simulink model "backflow_test"  (R2024b)
settings: Solver=FixedStepDiscrete  StartTime=0.0  StopTime=600  FixedStep=0.0002  RelTol=1e-3
InitFcn:
  |    parameters_charlton;
  |    parameters_ferreira;
  |    parameters_backflowcontrol;
undefined symbols (not defined in the file): A_tank, DiscIntNeverNeededParam, H_REF_MAX, H_REF_MIN, HR, Ki_fb, Kp_fb, LUT_Q, LUT_u, N, Ts, U_FB_MAX
libraries: slpidlib x2, simulink x1
settings Model: Creator=sammy  LastModifiedBy=sammy

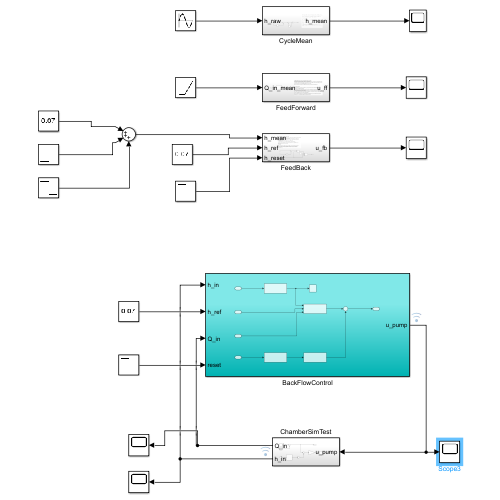
[thumbnail: Simulink's stored preview of the top-level diagram]
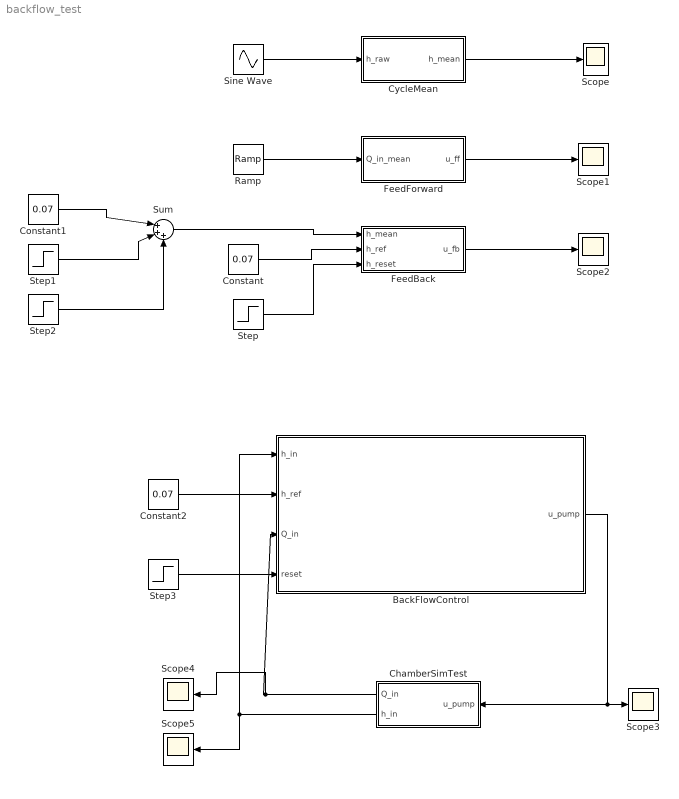
== system backflow_test ==
  BackFlowControl : Subsystem
  ChamberSimTest : Subsystem
  Constant : Constant  Value=0.07
  Constant1 : Constant  Value=0.07
  Constant2 : Constant  Value=0.07
  CycleMean : Subsystem
  FeedBack : Subsystem
  FeedForward : Subsystem
  Ramp : simulink/Sources/Ramp  slope=10  start=0  InitialOutput=0
  Scope{,1..5} (6 alike) : Scope
  Sine Wave : Sin  Amplitude=10  Frequency=2*pi*HR/60  SampleTime=0
  Step : Step  Time=5  Before=1  After=0  SampleTime=0
  Step1 : Step  Time=10  After=0.02  SampleTime=0
  Step2 : Step  Time=70  After=-0.02  SampleTime=0
  Step3 : Step  Time=5  Before=1  After=0  SampleTime=0
  Sum : Sum  Inputs=|+++
  wires:
  Sine Wave/1 -> CycleMean/1(h_raw)
  CycleMean/1(h_mean) -> Scope/1
  Ramp/1 -> FeedForward/1(Q_in_mean)
  FeedForward/1(u_ff) -> Scope1/1
  Step/1 -> FeedBack/3(h_reset)
  Constant/1 -> FeedBack/2(h_ref)
  Sum/1 -> FeedBack/1(h_mean)
  Constant1/1 -> Sum/1
  Step1/1 -> Sum/2
  Step2/1 -> Sum/3
  FeedBack/1(u_fb) -> Scope2/1
  BackFlowControl/1(u_pump) -> Scope3/1, ChamberSimTest/1(u_pump)
  ChamberSimTest/2(h_in) -> Scope5/1, BackFlowControl/1(h_in)
  Constant2/1 -> BackFlowControl/2(h_ref)
  Step3/1 -> BackFlowControl/4(reset)
  ChamberSimTest/1(Q_in) -> Scope4/1, BackFlowControl/3(Q_in)

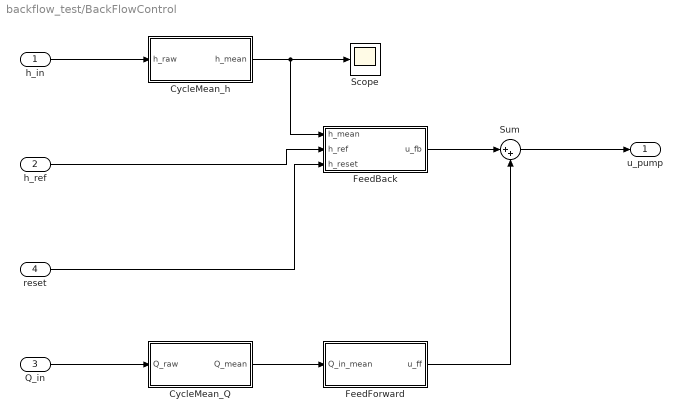
== system backflow_test/BackFlowControl ==
  h_in : Inport  SampleTime=Ts
  h_ref : Inport  Port=2  SampleTime=Ts
  Q_in : Inport  Port=3  SampleTime=Ts
  reset : Inport  Port=4  SampleTime=Ts
  CycleMean_Q : Subsystem
  CycleMean_h : Subsystem
  FeedBack : Subsystem
  FeedForward : Subsystem
  Scope : Scope
  Sum : Sum  Inputs=|++
  u_pump : Outport
  wires:
  Sum/1 -> u_pump/1
  h_in/1 -> CycleMean_h/1(h_raw)
  CycleMean_h/1(h_mean) -> Scope/1, FeedBack/1(h_mean)
  Q_in/1 -> CycleMean_Q/1(Q_raw)
  CycleMean_Q/1(Q_mean) -> FeedForward/1(Q_in_mean)
  h_ref/1 -> FeedBack/2(h_ref)
  reset/1 -> FeedBack/3(h_reset)
  FeedBack/1(u_fb) -> Sum/1
  FeedForward/1(u_ff) -> Sum/2

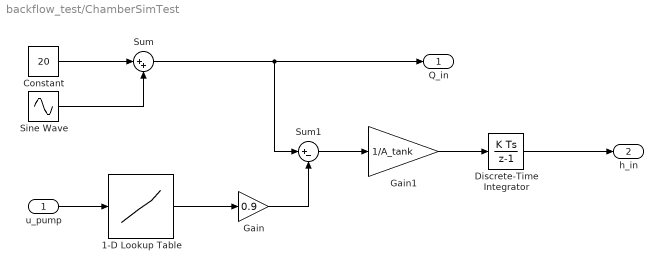
== system backflow_test/ChamberSimTest ==
  u_pump : Inport
  1-D Lookup Table : Lookup_n-D  NumberOfTableDimensions=1  BreakpointsForDimension1=LUT_u  Table=LUT_Q  ExtrapMethod=Clip  InternalRulePriority=Speed  RndMeth=Simplest
  Constant : Constant  Value=20
  Discrete-Time Integrator : DiscreteIntegrator  InitialCondition=0.07  SampleTime=Ts  ICPrevOutput=DiscIntNeverNeededParam  ICPrevScaledInput=DiscIntNeverNeededParam
  Gain : Gain  Gain=0.9
  Gain1 : Gain  Gain=1/A_tank
  Sine Wave : Sin  Amplitude=15  Frequency=2*pi*HR/60  SampleTime=Ts
  Sum : Sum  Inputs=|++
  Sum1 : Sum  Inputs=|+-
  Q_in : Outport
  h_in : Outport  Port=2
  wires:
  Constant/1 -> Sum/1
  Sine Wave/1 -> Sum/2
  Sum/1 -> Sum1/1, Q_in/1
  u_pump/1 -> 1-D Lookup Table/1
  1-D Lookup Table/1 -> Gain/1
  Gain/1 -> Sum1/2
  Sum1/1 -> Gain1/1
  Gain1/1 -> Discrete-Time Integrator/1
  Discrete-Time Integrator/1 -> h_in/1

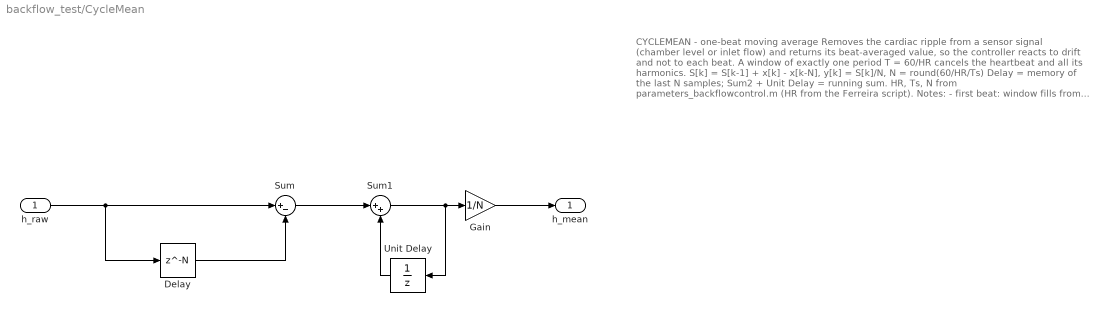
== system backflow_test/CycleMean ==
  note: CYCLEMEAN - one-beat moving average
      |
      | Removes the cardiac ripple from a sensor signal (chamber level or inlet flow) and returns its beat-averaged value, so the controller reacts to drift and not to each beat. A window of exactly one period T = 60/HR cancels the heartbeat and all its harmonics.
      |
      | S[k] = S[k-1] + x[k] - x[k-N], y[k] = S[k]/N,
      | N = round(60/HR/Ts)
      | Delay = memory of the last N samples; Sum2 + Unit Delay = running sum.
      |
      | HR, Ts, N from parameters_backflowcontrol.m (HR from the Ferreira script).
      | Notes:
      | - first beat: window fills from zero, output not valid before t = 60/HR
      | - input must run at Ts (enforced on the Inport)
      | - HR must match the generator, otherwise a residual ripple remains
      | - Delay and Unit Delay initial conditions must stay consistent
  h_raw : Inport
  Delay : Delay  DelayLength=N
  Gain : Gain  Gain=1/N
  Sum : Sum  Inputs=|+-
  Sum1 : Sum  Inputs=|++
  Unit Delay : UnitDelay  SampleTime=-1  HasFrameUpgradeWarning=on
  h_mean : Outport
  wires:
  h_raw/1 -> Sum/1, Delay/1
  Delay/1 -> Sum/2
  Sum/1 -> Sum1/1
  Sum1/1 -> Unit Delay/1, Gain/1
  Gain/1 -> h_mean/1
  Unit Delay/1 -> Sum1/2

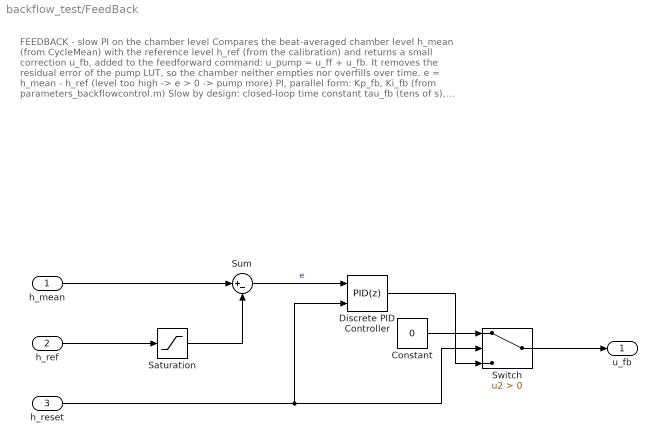
== system backflow_test/FeedBack ==
  note: FEEDBACK - slow PI on the chamber level
      | Compares the beat-averaged chamber level h_mean (from CycleMean) with the reference level h_ref (from the calibration) and returns a small correction u_fb, added to the feedforward command: u_pump = u_ff + u_fb.
      | It removes the residual error of the pump LUT, so the chamber neither empties nor overfills over time.
      | e = h_mean - h_ref (level too high -> e > 0 -> pump more)
      | PI, parallel form: Kp_fb, Ki_fb (from parameters_backflowcontrol.m)
      | Slow by design: closed-loop time constant tau_fb (tens of s), integral time Ti_fb = 4*tau_fb.
      | The feedforward does most of the work.
      | Protections:
      | - h_ref saturated to [H_REF_MIN, H_REF_MAX]: never track an absurd setpoint
      | - output limited to +/- U_FB_MAX (limited authority), clamping anti-windup
      | - reset = 1 (during calibration): integrator held at 0 and u_fb = 0, pump runs on feedforward only
  h_mean : Inport  SampleTime=Ts
  h_ref : Inport  Port=2  SampleTime=Ts
  h_reset : Inport  Port=3  SampleTime=Ts
  Constant : Constant  Value=0
  Discrete PID Controller : slpidlib/PID Controller  Controller=PID  Form=Parallel  TimeDomain=Discrete-time  UseExternalTs=off  SampleTime=Ts  IntegratorMethod=Forward Euler  FilterMethod=Forward Euler  ControllerParametersSource=internal  P=Kp_fb  I=Ki_fb  UseKiTs=off  D=0  UseExternalDerivativeSource=off  N=100  UseFilter=on  TunerSelectOption=Transfer Function Based (PID Tuner App)  InitialConditionSource=internal  InitialConditionForIntegrator=0  InitialConditionForFilter=0  DifferentiatorICPrevScaledInput=0  ExternalReset=level  TrackingMode=off  Kt=1  LimitOutput=on  SatLimitsSource=internal  UpperSaturationLimit=U_FB_MAX  LowerSaturationLimit=-U_FB_MAX  LinearizeAsGain=off  AntiWindupMode=clamping  Kb=1  LimitIntegrator=off  UpperIntegratorSaturationLimit=inf  LowerIntegratorSaturationLimit=-inf  POutMin=[]  POutMax=[]  IOutMin=[]  IOutMax=[]  DOutMin=[]  DOutMax=[]  NOutMin=[]  NOutMax=[]  SumOutMin=[]  SumOutMax=[]  SaturationOutMin=[]  SaturationOutMax=[]  PParamMin=[]  PParamMax=[]  IParamMin=[]  IParamMax=[]  DParamMin=[]  DParamMax=[]  NParamMin=[]  NParamMax=[]  KbParamMin=[]  KbParamMax=[]  KtParamMin=[]  KtParamMax=[]  KbOutMin=[]  KbOutMax=[]  KtOutMin=[]  KtOutMax=[]  IntegratorOutMin=[]  IntegratorOutMax=[]  FilterOutMin=[]  FilterOutMax=[]  SumI1OutMin=[]  SumI1OutMax=[]  SumI2OutMin=[]  SumI2OutMax=[]  SumI3OutMin=[]  SumI3OutMax=[]  SumI4OutMin=[]  SumI4OutMax=[]  SumDOutMin=[]  SumDOutMax=[]  DifferentiatorOutMin=[]  DifferentiatorOutMax=[]  FilterDiffOutCoefMin=[]  FilterDiffOutCoefMax=[]  ReciprocalOutMin=[]  ReciprocalOutMax=[]  SumDenOutMin=[]  SumDenOutMax=[]  SumNumOutMin=[]  SumNumOutMax=[]  DivideOutMin=[]  DivideOutMax=[]  UdiffTsProdOutMin=[]  UdiffTsProdOutMax=[]  NTsProdOutMin=[]  NTsProdOutMax=[]  UintegralTsProdOutMin=[]  UintegralTsProdOutMax=[]  UngainTsProdOutMin=[]  UngainTsProdOutMax=[]  ClampingZeroOutDataTypeStr=Inherit: Inherit via back propagation  ClampingZeroOutMin=[]  ClampingZeroOutMax=[]  FilterDenConstantOutDataTypeStr=Inherit: Inherit via back propagation  FilterDenConstantOutMin=[]  FilterDenConstantOutMax=[]  PCopyOutDataTypeStr=Inherit: Inherit via back propagation  PCopyOutMin=[]  PCopyOutMax=[]  NCopyOutDataTypeStr=Inherit: Inherit via back propagation  NCopyOutMin=[]  NCopyOutMax=[]  IntegratorContinuousStateAttributes=''  IntegratorStateMustResolveToSignalObject=off  IntegratorRTWStateStorageClass=Auto  FilterContinuousStateAttributes=''  FilterStateMustResolveToSignalObject=off  FilterRTWStateStorageClass=Auto  ParallelPVariant=InternalParameters  IdealPVariant=Disabled  IVariant=InternalParameters  DVariant=InternalParameters  IntegratorVariant=Discrete  SatVariant=Enabled  AWVariant=DiscClampingParallel  PCopyVariant=Disabled  TRVariant=Disabled  FdbkBlocksVariant=Forward  IdealPFdbkVariant=Disabled  SatFdbkVariant=Disabled  DerivativeFilterVariant=ForwardEulerFilter  NVariant=InternalParameters  NCopyVariant=Disabled  FilterICVariant=InternalICsFilter  IntegratorICVariant=InternalICs  ExternalResetVariant=ExternalReset  TRSumVariant=Passthrough  SumFdbkVariant=Disabled  SumVariant=Sum_PID  TsampFilterVariant=InternalTs  TsampNgainVariant=Passthrough  TsampIntegralVariant=Disabled_SignalSpec  ExternalSaturationOutDataTypeStr=Inherit: Same as second input  DerivativeSourceVariant=ErrorSignal  PreIntVariant=InternalPreInt
      settings: LibrarySourceBlock=simulink/Discrete/Discrete PID Controller
  Saturation : Saturate  UpperLimit=H_REF_MAX  LowerLimit=H_REF_MIN
  Sum : Sum  Inputs=|+-
  Switch : Switch  Criteria=u2 > Threshold  SaturateOnIntegerOverflow=off  InputSameDT=off
  u_fb : Outport
  wires:
  h_ref/1 -> Saturation/1
  Saturation/1 -> Sum/2
  h_mean/1 -> Sum/1
  Sum/1 -> Discrete PID Controller/1  "e"
  h_reset/1 -> Switch/2, Discrete PID Controller/2
  Discrete PID Controller/1 -> Switch/3
  Constant/1 -> Switch/1
  Switch/1 -> u_fb/1

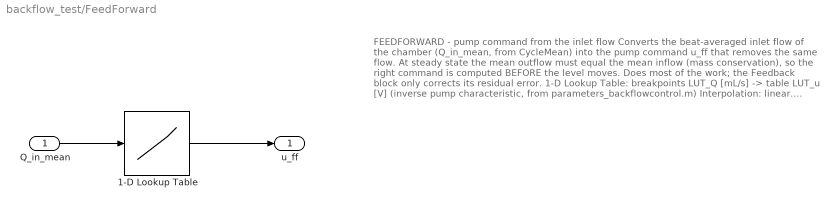
== system backflow_test/FeedForward ==
  note: FEEDFORWARD - pump command from the inlet flow
      | Converts the beat-averaged inlet flow of the chamber (Q_in_mean, from CycleMean) into the pump command u_ff that removes the same flow.
      | At steady state the mean outflow must equal the mean inflow (mass conservation), so the right command is computed BEFORE the level moves.
      | Does most of the work; the Feedback block only corrects its residual error.
      |
      | 1-D Lookup Table:
      | breakpoints LUT_Q [mL/s] -> table LUT_u [V] (inverse pump characteristic, from parameters_backflowcontrol.m)
      | Interpolation: linear. Extrapolation: clip (no guess outside the measured range).
      | Uses the MEAN flow, not the instantaneous one: the chamber buffers the pulsatility, the pump only has to match the average.
      | LUT source selected in the script: LUT_SOURCE = 'mock' (test values) or 'measured' (Jabsco 23680-4103 in the real configuration).
      | Note: below the dead zone the interpolated command may be too low for the pump to actually run - to be handled with the measured curve.
  Q_in_mean : Inport  SampleTime=Ts
  1-D Lookup Table : Lookup_n-D  NumberOfTableDimensions=1  BreakpointsForDimension1=LUT_Q  Table=LUT_u  InterpMethod=Linear Lagrange  ExtrapMethod=Clip  InternalRulePriority=Speed  RndMeth=Simplest
  u_ff : Outport
  wires:
  Q_in_mean/1 -> 1-D Lookup Table/1
  1-D Lookup Table/1 -> u_ff/1

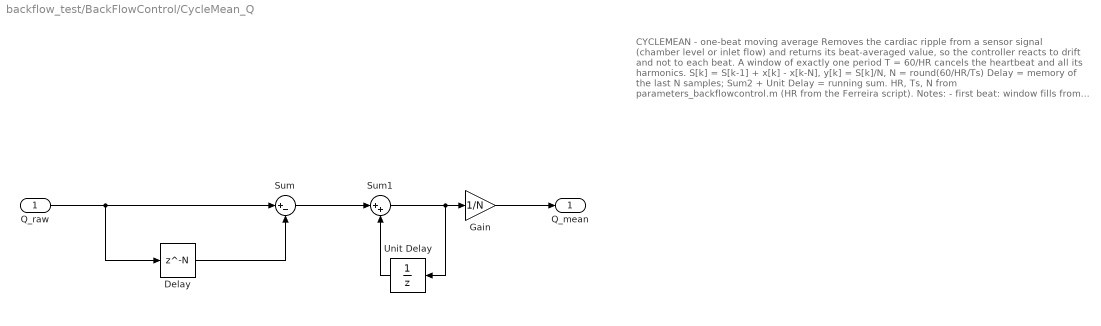
== system backflow_test/BackFlowControl/CycleMean_Q ==
  note: CYCLEMEAN - one-beat moving average
      |
      | Removes the cardiac ripple from a sensor signal (chamber level or inlet flow) and returns its beat-averaged value, so the controller reacts to drift and not to each beat. A window of exactly one period T = 60/HR cancels the heartbeat and all its harmonics.
      |
      | S[k] = S[k-1] + x[k] - x[k-N], y[k] = S[k]/N,
      | N = round(60/HR/Ts)
      | Delay = memory of the last N samples; Sum2 + Unit Delay = running sum.
      |
      | HR, Ts, N from parameters_backflowcontrol.m (HR from the Ferreira script).
      | Notes:
      | - first beat: window fills from zero, output not valid before t = 60/HR
      | - input must run at Ts (enforced on the Inport)
      | - HR must match the generator, otherwise a residual ripple remains
      | - Delay and Unit Delay initial conditions must stay consistent
  Q_raw : Inport
  Delay : Delay  DelayLength=N
  Gain : Gain  Gain=1/N
  Sum : Sum  Inputs=|+-
  Sum1 : Sum  Inputs=|++
  Unit Delay : UnitDelay  SampleTime=-1  HasFrameUpgradeWarning=on
  Q_mean : Outport
  wires:
  Q_raw/1 -> Sum/1, Delay/1
  Delay/1 -> Sum/2
  Sum/1 -> Sum1/1
  Sum1/1 -> Unit Delay/1, Gain/1
  Gain/1 -> Q_mean/1
  Unit Delay/1 -> Sum1/2

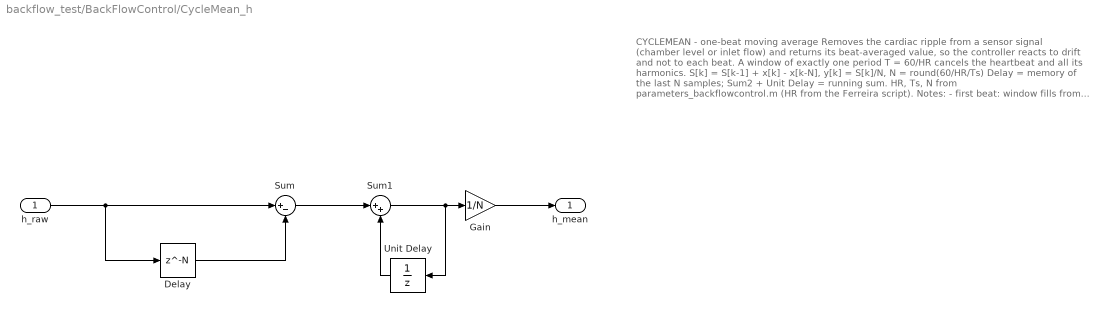
== system backflow_test/BackFlowControl/CycleMean_h ==
  note: CYCLEMEAN - one-beat moving average
      |
      | Removes the cardiac ripple from a sensor signal (chamber level or inlet flow) and returns its beat-averaged value, so the controller reacts to drift and not to each beat. A window of exactly one period T = 60/HR cancels the heartbeat and all its harmonics.
      |
      | S[k] = S[k-1] + x[k] - x[k-N], y[k] = S[k]/N,
      | N = round(60/HR/Ts)
      | Delay = memory of the last N samples; Sum2 + Unit Delay = running sum.
      |
      | HR, Ts, N from parameters_backflowcontrol.m (HR from the Ferreira script).
      | Notes:
      | - first beat: window fills from zero, output not valid before t = 60/HR
      | - input must run at Ts (enforced on the Inport)
      | - HR must match the generator, otherwise a residual ripple remains
      | - Delay and Unit Delay initial conditions must stay consistent
  h_raw : Inport
  Delay : Delay  DelayLength=N
  Gain : Gain  Gain=1/N
  Sum : Sum  Inputs=|+-
  Sum1 : Sum  Inputs=|++
  Unit Delay : UnitDelay  SampleTime=-1  HasFrameUpgradeWarning=on
  h_mean : Outport
  wires:
  h_raw/1 -> Sum/1, Delay/1
  Delay/1 -> Sum/2
  Sum/1 -> Sum1/1
  Sum1/1 -> Unit Delay/1, Gain/1
  Gain/1 -> h_mean/1
  Unit Delay/1 -> Sum1/2

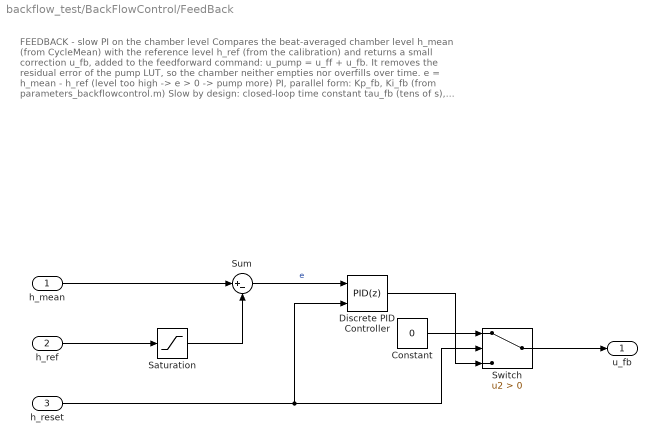
== system backflow_test/BackFlowControl/FeedBack ==
  note: FEEDBACK - slow PI on the chamber level
      | Compares the beat-averaged chamber level h_mean (from CycleMean) with the reference level h_ref (from the calibration) and returns a small correction u_fb, added to the feedforward command: u_pump = u_ff + u_fb.
      | It removes the residual error of the pump LUT, so the chamber neither empties nor overfills over time.
      | e = h_mean - h_ref (level too high -> e > 0 -> pump more)
      | PI, parallel form: Kp_fb, Ki_fb (from parameters_backflowcontrol.m)
      | Slow by design: closed-loop time constant tau_fb (tens of s), integral time Ti_fb = 4*tau_fb.
      | The feedforward does most of the work.
      | Protections:
      | - h_ref saturated to [H_REF_MIN, H_REF_MAX]: never track an absurd setpoint
      | - output limited to +/- U_FB_MAX (limited authority), clamping anti-windup
      | - reset = 1 (during calibration): integrator held at 0 and u_fb = 0, pump runs on feedforward only
  h_mean : Inport  SampleTime=Ts
  h_ref : Inport  Port=2  SampleTime=Ts
  h_reset : Inport  Port=3  SampleTime=Ts
  Constant : Constant  Value=0
  Discrete PID Controller : slpidlib/PID Controller  Controller=PID  Form=Parallel  TimeDomain=Discrete-time  UseExternalTs=off  SampleTime=Ts  IntegratorMethod=Forward Euler  FilterMethod=Forward Euler  ControllerParametersSource=internal  P=Kp_fb  I=Ki_fb  UseKiTs=off  D=0  UseExternalDerivativeSource=off  N=100  UseFilter=on  TunerSelectOption=Transfer Function Based (PID Tuner App)  InitialConditionSource=internal  InitialConditionForIntegrator=0  InitialConditionForFilter=0  DifferentiatorICPrevScaledInput=0  ExternalReset=level  TrackingMode=off  Kt=1  LimitOutput=on  SatLimitsSource=internal  UpperSaturationLimit=U_FB_MAX  LowerSaturationLimit=-U_FB_MAX  LinearizeAsGain=off  AntiWindupMode=clamping  Kb=1  LimitIntegrator=off  UpperIntegratorSaturationLimit=inf  LowerIntegratorSaturationLimit=-inf  POutMin=[]  POutMax=[]  IOutMin=[]  IOutMax=[]  DOutMin=[]  DOutMax=[]  NOutMin=[]  NOutMax=[]  SumOutMin=[]  SumOutMax=[]  SaturationOutMin=[]  SaturationOutMax=[]  PParamMin=[]  PParamMax=[]  IParamMin=[]  IParamMax=[]  DParamMin=[]  DParamMax=[]  NParamMin=[]  NParamMax=[]  KbParamMin=[]  KbParamMax=[]  KtParamMin=[]  KtParamMax=[]  KbOutMin=[]  KbOutMax=[]  KtOutMin=[]  KtOutMax=[]  IntegratorOutMin=[]  IntegratorOutMax=[]  FilterOutMin=[]  FilterOutMax=[]  SumI1OutMin=[]  SumI1OutMax=[]  SumI2OutMin=[]  SumI2OutMax=[]  SumI3OutMin=[]  SumI3OutMax=[]  SumI4OutMin=[]  SumI4OutMax=[]  SumDOutMin=[]  SumDOutMax=[]  DifferentiatorOutMin=[]  DifferentiatorOutMax=[]  FilterDiffOutCoefMin=[]  FilterDiffOutCoefMax=[]  ReciprocalOutMin=[]  ReciprocalOutMax=[]  SumDenOutMin=[]  SumDenOutMax=[]  SumNumOutMin=[]  SumNumOutMax=[]  DivideOutMin=[]  DivideOutMax=[]  UdiffTsProdOutMin=[]  UdiffTsProdOutMax=[]  NTsProdOutMin=[]  NTsProdOutMax=[]  UintegralTsProdOutMin=[]  UintegralTsProdOutMax=[]  UngainTsProdOutMin=[]  UngainTsProdOutMax=[]  ClampingZeroOutDataTypeStr=Inherit: Inherit via back propagation  ClampingZeroOutMin=[]  ClampingZeroOutMax=[]  FilterDenConstantOutDataTypeStr=Inherit: Inherit via back propagation  FilterDenConstantOutMin=[]  FilterDenConstantOutMax=[]  PCopyOutDataTypeStr=Inherit: Inherit via back propagation  PCopyOutMin=[]  PCopyOutMax=[]  NCopyOutDataTypeStr=Inherit: Inherit via back propagation  NCopyOutMin=[]  NCopyOutMax=[]  IntegratorContinuousStateAttributes=''  IntegratorStateMustResolveToSignalObject=off  IntegratorRTWStateStorageClass=Auto  FilterContinuousStateAttributes=''  FilterStateMustResolveToSignalObject=off  FilterRTWStateStorageClass=Auto  ParallelPVariant=InternalParameters  IdealPVariant=Disabled  IVariant=InternalParameters  DVariant=InternalParameters  IntegratorVariant=Discrete  SatVariant=Enabled  AWVariant=DiscClampingParallel  PCopyVariant=Disabled  TRVariant=Disabled  FdbkBlocksVariant=Forward  IdealPFdbkVariant=Disabled  SatFdbkVariant=Disabled  DerivativeFilterVariant=ForwardEulerFilter  NVariant=InternalParameters  NCopyVariant=Disabled  FilterICVariant=InternalICsFilter  IntegratorICVariant=InternalICs  ExternalResetVariant=ExternalReset  TRSumVariant=Passthrough  SumFdbkVariant=Disabled  SumVariant=Sum_PID  TsampFilterVariant=InternalTs  TsampNgainVariant=Passthrough  TsampIntegralVariant=Disabled_SignalSpec  ExternalSaturationOutDataTypeStr=Inherit: Same as second input  DerivativeSourceVariant=ErrorSignal  PreIntVariant=InternalPreInt
  Saturation : Saturate  UpperLimit=H_REF_MAX  LowerLimit=H_REF_MIN
  Sum : Sum  Inputs=|+-
  Switch : Switch  Criteria=u2 > Threshold  SaturateOnIntegerOverflow=off  InputSameDT=off
  u_fb : Outport
  wires:
  h_ref/1 -> Saturation/1
  Saturation/1 -> Sum/2
  h_mean/1 -> Sum/1
  Sum/1 -> Discrete PID Controller/1  "e"
  h_reset/1 -> Switch/2, Discrete PID Controller/2
  Discrete PID Controller/1 -> Switch/3
  Constant/1 -> Switch/1
  Switch/1 -> u_fb/1

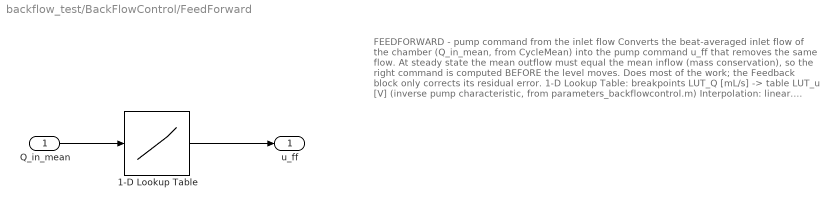
== system backflow_test/BackFlowControl/FeedForward ==
  note: FEEDFORWARD - pump command from the inlet flow
      | Converts the beat-averaged inlet flow of the chamber (Q_in_mean, from CycleMean) into the pump command u_ff that removes the same flow.
      | At steady state the mean outflow must equal the mean inflow (mass conservation), so the right command is computed BEFORE the level moves.
      | Does most of the work; the Feedback block only corrects its residual error.
      |
      | 1-D Lookup Table:
      | breakpoints LUT_Q [mL/s] -> table LUT_u [V] (inverse pump characteristic, from parameters_backflowcontrol.m)
      | Interpolation: linear. Extrapolation: clip (no guess outside the measured range).
      | Uses the MEAN flow, not the instantaneous one: the chamber buffers the pulsatility, the pump only has to match the average.
      | LUT source selected in the script: LUT_SOURCE = 'mock' (test values) or 'measured' (Jabsco 23680-4103 in the real configuration).
      | Note: below the dead zone the interpolated command may be too low for the pump to actually run - to be handled with the measured curve.
  Q_in_mean : Inport  SampleTime=Ts
  1-D Lookup Table : Lookup_n-D  NumberOfTableDimensions=1  BreakpointsForDimension1=LUT_Q  Table=LUT_u  InterpMethod=Linear Lagrange  ExtrapMethod=Clip  InternalRulePriority=Speed  RndMeth=Simplest
  u_ff : Outport
  wires:
  Q_in_mean/1 -> 1-D Lookup Table/1
  1-D Lookup Table/1 -> u_ff/1
